simulink model "my_pendulum"  (R2023b)
settings: Solver=VariableStepAuto  StartTime=0.0  StopTime=10.0  MaxStep=0.01  RelTol=1e-3
values from neighbouring files (symbols this model uses):
  I = m*L^2    [pendulum_mask.m]
libraries: simulink_extras x3
settings Model: Creator=user  LastModifiedBy=user

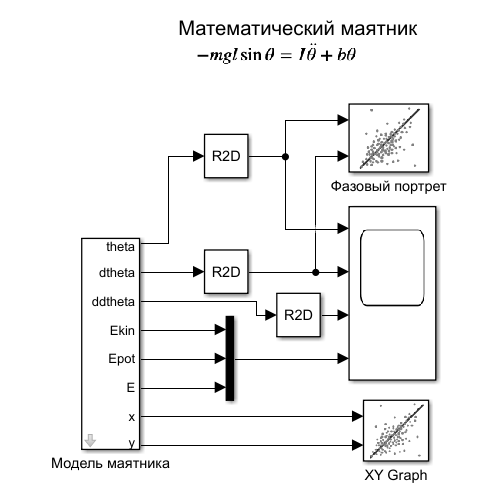
[thumbnail: Simulink's stored preview of the top-level diagram]
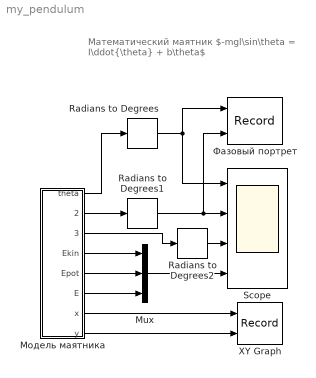
== system my_pendulum ==
  note: Математический маятник
      | $-mgl\sin\theta = I\ddot{\theta} + b\theta$
  Mux : Mux  Inputs=3
  Radians to Degrees : simulink_extras/Transformations/Radians to Degrees
  Radians to Degrees1 : simulink_extras/Transformations/Radians to Degrees
  Radians to Degrees2 : simulink_extras/Transformations/Radians to Degrees
  Scope : Scope  NumInputPorts=4
  XY Graph : Record  FileSettingsInternal="{\"entries\":[{\"content\":{\"excelSettings\":{\"content\":{},\"type\":\"Streamout.ExcelSettings\"}},\"type\":\"Streamout.FileSettingStorage\",\"uuid\":\"\"}],\"packageUris\":[\"http:\\/\\/schema.mathworks.com\\/mf0\\/streamout_blocks\\/R2020a\"],\"version\":\"1.0\"}"  Layout=[1 1]  SignalsInternal="{\"entries\":[{\"content\":{\"signals\":[{\"content\":{\"blockPath\":[],\"dimensions\":[1],\"domain\":\"\",\"lineColor\":\"#a2142f\",\"plots\":[1],\"port\":1,\"sid\":[\"\"],\"signalID\":74,\"signalName\":\"Модель маятника:7\"},\"type\":\"RecordBlkView.Signal\",\"uuid\":\"\"},{\"content\":{\"blockPath\":[],\"dimensions\":[1],\"domain\":\"\",\"lineColor\":\"#139fff\",\"plots\":[1],\"port\":2,\"sid\":[\"\"],\"signalID\":78,\"signalName\":\"Модель маятника:8\"},\"type\":\"RecordBlkView.Signal\",\"uuid\":\"\"}]},\"type\":\"RecordBlkView.InputSignals\",\"uuid\":\"\"}],\"packageUris\":[\"http:\\/\\/schema.mathworks.com\\/mf0\\/streamout_blocks\\/R2020a\"],\"version\":\"1.0\"}"  VisualizationBindings="{\"xyplotplugin\":{\"info\":[{\"series\":[{\"bindingParametersList\":[{\"parameter\":\"X-Axis\",\"signalID\":74,\"signalName\":\"Модель маятника:7\"},{\"parameter\":\"Y-Axis\",\"signalID\":78,\"signalName\":\"Модель маятника:8\"}],\"seriesID\":51814}],\"subplotID\":1}]}}"  CompatibilityTag=XY
  Модель маятника : Subsystem  mask{m=1, g=9.8, L=1, start_theta=30, b=0.03}
      mask prompts: m "Масса"; g "Ускорение св. падения"; L "Длина подвеса"; start_theta "Стартовый угол"; b "Коэффициент диссипации"
  Фазовый портрет : Record  FileSettingsInternal="{\"entries\":[{\"content\":{\"excelSettings\":{\"content\":{},\"type\":\"Streamout.ExcelSettings\"}},\"type\":\"Streamout.FileSettingStorage\",\"uuid\":\"\"}],\"packageUris\":[\"http:\\/\\/schema.mathworks.com\\/mf0\\/streamout_blocks\\/R2020a\"],\"version\":\"1.0\"}"  Layout=[1 1]  SignalsInternal="{\"entries\":[{\"content\":{\"signals\":[{\"content\":{\"blockPath\":[],\"dimensions\":[1],\"domain\":\"\",\"lineColor\":\"#a2142f\",\"plots\":[1],\"port\":1,\"sid\":[\"\"],\"signalID\":82,\"signalName\":\"Radians\\nto Degrees\"},\"type\":\"RecordBlkView.Signal\",\"uuid\":\"\"},{\"content\":{\"blockPath\":[],\"dimensions\":[1],\"domain\":\"\",\"lineColor\":\"#139fff\",\"plots\":[1],\"port\":2,\"sid\":[\"\"],\"signalID\":86,\"signalName\":\"Radians\\nto Degrees1\"},\"type\":\"RecordBlkView.Signal\",\"uuid\":\"\"}]},\"type\":\"RecordBlkView.InputSignals\",\"uuid\":\"\"}],\"packageUris\":[\"http:\\/\\/schema.mathworks.com\\/mf0\\/streamout_blocks\\/R2020a\"],\"version\":\"1.0\"}"  VisualizationBindings="{\"xyplotplugin\":{\"info\":[{\"series\":[{\"bindingParametersList\":[{\"parameter\":\"X-Axis\",\"signalID\":82,\"signalName\":\"Radians\\nto Degrees\"},{\"parameter\":\"Y-Axis\",\"signalID\":86,\"signalName\":\"Radians\\nto Degrees1\"}],\"seriesID\":8943}],\"subplotID\":1}]}}"  CompatibilityTag=XY
  wires:
  Модель маятника/4(Ekin) -> Mux/1
  Модель маятника/5(Epot) -> Mux/2
  Модель маятника/6(E) -> Mux/3
  Mux/1 -> Scope/4
  Модель маятника/1(theta) -> Radians to Degrees/1
  Модель маятника/2(dtheta) -> Radians to Degrees1/1
  Модель маятника/7(x) -> XY Graph/1
  Модель маятника/8(y) -> XY Graph/2
  Radians to Degrees/1 -> Scope/1, Фазовый портрет/1
  Radians to Degrees1/1 -> Фазовый портрет/2, Scope/2
  Radians to Degrees2/1 -> Scope/3
  Модель маятника/3(ddtheta) -> Radians to Degrees2/1

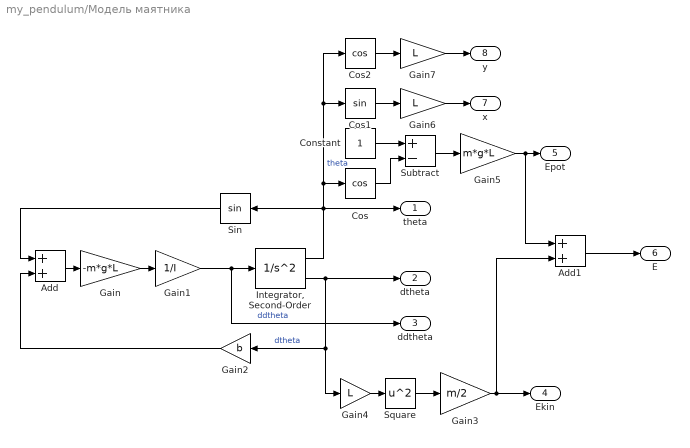
== system my_pendulum/Модель маятника ==
  Add : Sum
  Add1 : Sum
  Constant : Constant
  Cos : Trigonometry  Operator=cos
  Cos1 : Trigonometry
  Cos2 : Trigonometry  Operator=cos
  Gain : Gain  Gain=-m*g*L
  Gain1 : Gain  Gain=1/I
  Gain2 : Gain  Gain=b
  Gain3 : Gain  Gain=m/2
  Gain4 : Gain  Gain=L
  Gain5 : Gain  Gain=m*g*L
  Gain6 : Gain  Gain=L
  Gain7 : Gain  Gain=L
  "Integrator, Second-Order" : SecondOrderIntegrator  ICX=deg2rad(start_theta)
  Sin : Trigonometry
  Square : Math  Operator=square
  Subtract : Sum  Inputs=+-
  theta : Outport
  dtheta : Outport  Port=2
  ddtheta : Outport  Port=3
  Ekin : Outport  Port=4
  Epot : Outport  Port=5
  E : Outport  Port=6
  x : Outport  Port=7
  y : Outport  Port=8
  wires:
  "Integrator, Second-Order"/2 -> Gain4/1, Gain2/1, dtheta/1  "dtheta"
  Sin/1 -> Add/1
  Gain/1 -> Gain1/1
  Gain1/1 -> ddtheta/1, "Integrator, Second-Order"/1  "ddtheta"
  "Integrator, Second-Order"/1 -> Cos2/1, Cos1/1, Cos/1, theta/1, Sin/1  "theta"
  Gain2/1 -> Add/2
  Add/1 -> Gain/1
  Square/1 -> Gain3/1
  Gain4/1 -> Square/1
  Gain3/1 -> Add1/2, Ekin/1
  Add1/1 -> E/1
  Cos1/1 -> Gain6/1
  Gain6/1 -> x/1
  Gain7/1 -> y/1
  Cos2/1 -> Gain7/1
  Constant/1 -> Subtract/1
  Cos/1 -> Subtract/2
  Subtract/1 -> Gain5/1
  Gain5/1 -> Add1/1, Epot/1
